simulink model "three_tank_open_loop"  (R2025b)
settings: Solver=ode4  StartTime=0.0  StopTime=20000  FixedStep=0.5  RelTol=1e-3
settings Model: Creator=user  LastModifiedBy=USER PC

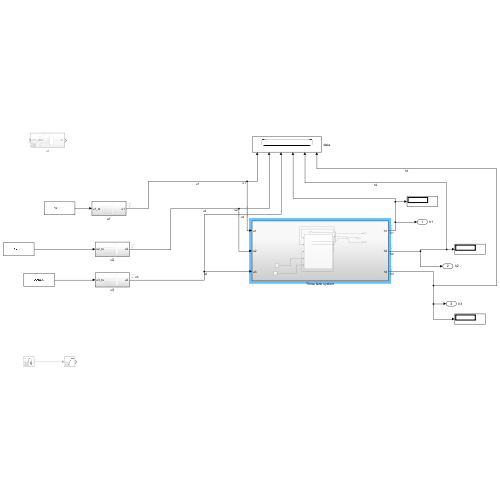
[thumbnail: Simulink's stored preview of the top-level diagram]
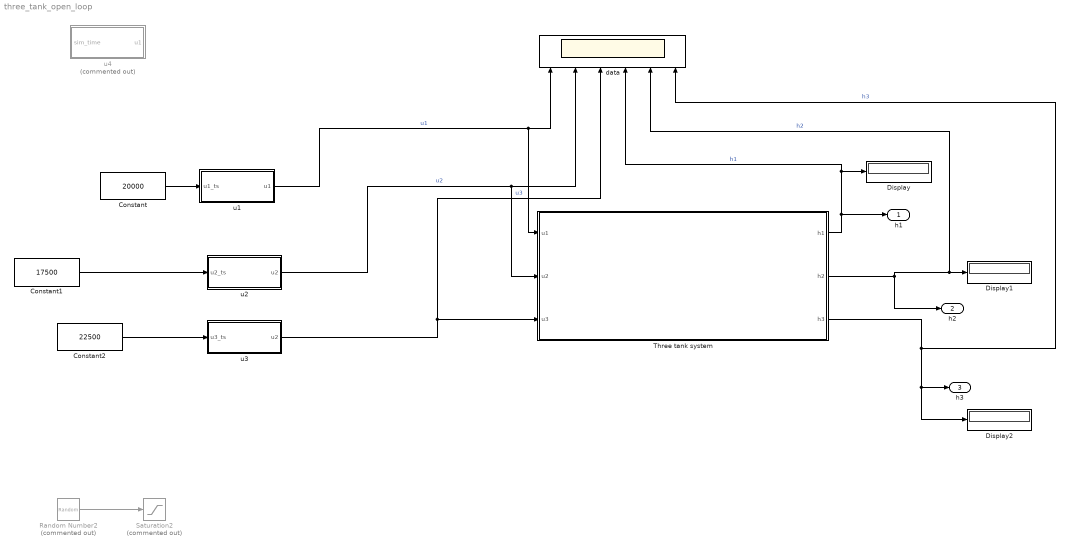
== system three_tank_open_loop ==
  Constant : Constant  Value=20000
  Constant1 : Constant  Value=17500
  Constant2 : Constant  Value=22500
  Display : Display
  Display1 : Display
  Display2 : Display
  Random Number2 : RandomNumber  Commented=on  Mean=0.2  Variance=0.01  Seed=1600  SampleTime=50
  Saturation2 : Saturate  Commented=on  UpperLimit=0.4  LowerLimit=0.01
  Three tank system : Subsystem
  data : Scope  NumInputPorts=6
      settings: ActiveDisplayString=5  Title=Tank 2 Height  ShowGrid=off  ActiveDisplayYMinimum=-4.7717687691549289  ActiveDisplayYMaximum=43.084803886371247  YLabel=Height (cm)  DataLoggingVariableName=dataset
  u1 : Subsystem
  u2 : Subsystem
  u3 : Subsystem
  u4 : Subsystem  Commented=on
  h1 : Outport
  h2 : Outport  Port=2
  h3 : Outport  Port=3
  wires:
  u3/1(u2) -> data/3, Three tank system/3(u3)  "u3"
  u2/1(u2) -> data/2, Three tank system/2(u2)  "u2"
  u1/1(u1) -> Three tank system/1(u1), data/1  "u1"
  Three tank system/3(h3) -> Display2/1, h3/1, data/6  "h3"
  Three tank system/2(h2) -> Display1/1, data/5, h2/1  "h2"
  Random Number2/1 -> Saturation2/1
  Three tank system/1(h1) -> h1/1, data/4, Display/1  "h1"
  Constant/1 -> u1/1(u1_ts)
  Constant1/1 -> u2/1(u2_ts)
  Constant2/1 -> u3/1(u3_ts)

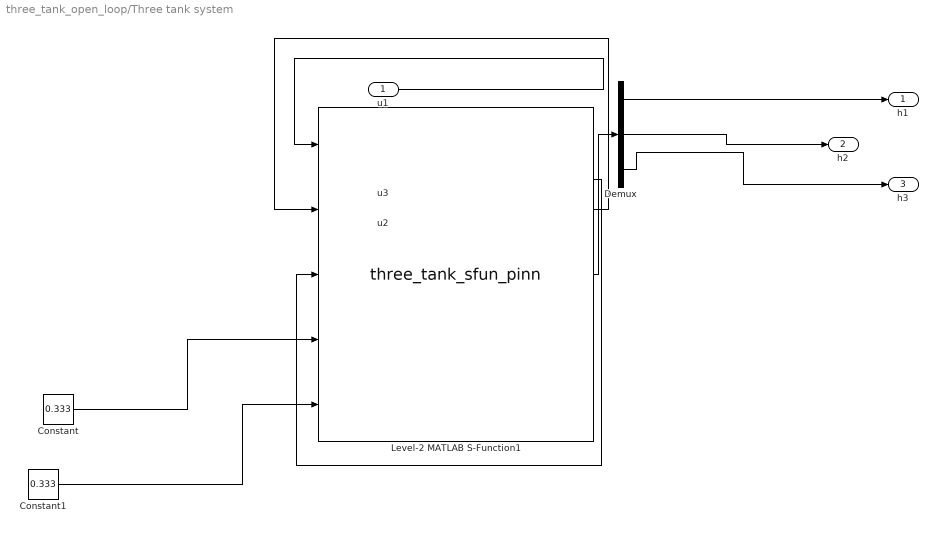
== system three_tank_open_loop/Three tank system ==
  u1 : Inport
  u2 : Inport  Port=2
  u3 : Inport  Port=3
  Constant : Constant  Value=0.333
  Constant1 : Constant  Value=0.333
  Demux : Demux  Outputs=3
  Level-2 MATLAB S-Function1 : M-S-Function  FunctionName=three_tank_sfun_pinn  Parameters=[5;5;5]
  h1 : Outport
  h2 : Outport  Port=2
  h3 : Outport  Port=3
  wires:
  u1/1 -> Level-2 MATLAB S-Function1/1
  u3/1 -> Level-2 MATLAB S-Function1/3
  u2/1 -> Level-2 MATLAB S-Function1/2
  Level-2 MATLAB S-Function1/1 -> Demux/1
  Demux/1 -> h1/1
  Demux/3 -> h3/1
  Demux/2 -> h2/1
  Constant/1 -> Level-2 MATLAB S-Function1/4
  Constant1/1 -> Level-2 MATLAB S-Function1/5

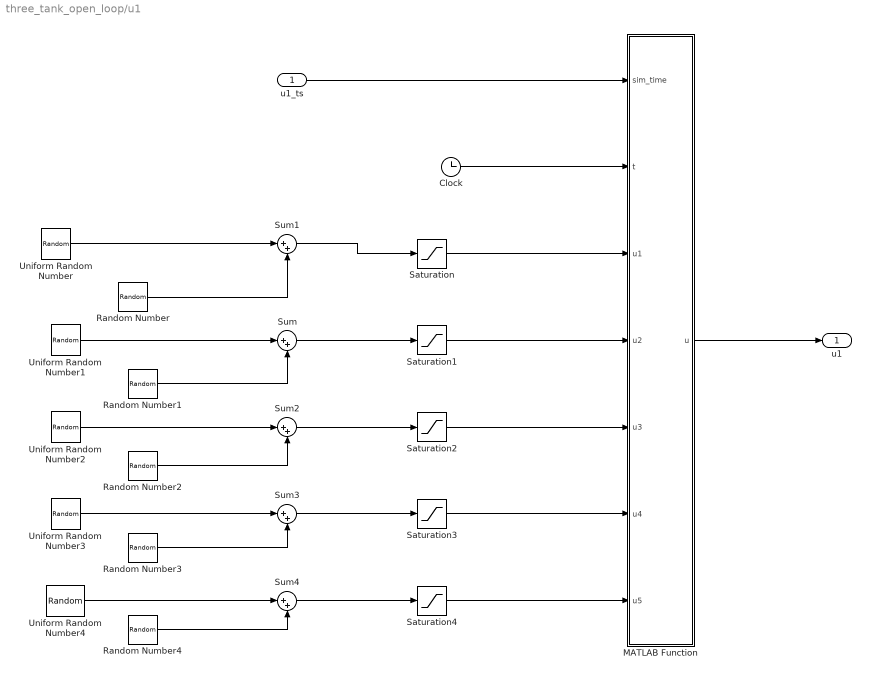
== system three_tank_open_loop/u1 ==
  u1_ts : Inport
  Clock : Clock
  MATLAB Function : MATLAB Function  TreatAsAtomicUnit=on
  Random Number : RandomNumber  Variance=0.05^2  Seed=122  SampleTime=1
  Random Number1 : RandomNumber  Variance=0.05^2  Seed=124  SampleTime=1
  Random Number2 : RandomNumber  Variance=0.05^2  Seed=126  SampleTime=1
  Random Number3 : RandomNumber  Variance=0.05^2  Seed=128  SampleTime=1
  Random Number4 : RandomNumber  Variance=0.05^2  Seed=130  SampleTime=1
  Saturation{,1..4} (5 alike) : Saturate  UpperLimit=148  LowerLimit=55
  Sum{,1..4} (5 alike) : Sum  Inputs=|++
  Uniform Random Number : UniformRandomNumber  Minimum=55  Maximum=148  Seed=121  SampleTime=20
  Uniform Random Number1 : UniformRandomNumber  Minimum=55  Maximum=148  Seed=123  SampleTime=40
  Uniform Random Number2 : UniformRandomNumber  Minimum=55  Maximum=148  Seed=125  SampleTime=60
  Uniform Random Number3 : UniformRandomNumber  Minimum=55  Maximum=148  Seed=127  SampleTime=80
  Uniform Random Number4 : UniformRandomNumber  Minimum=55  Maximum=148  Seed=129  SampleTime=100
  u1 : Outport
  wires:
  Clock/1 -> MATLAB Function/2(t)
  Saturation/1 -> MATLAB Function/3(u1)
  Saturation1/1 -> MATLAB Function/4(u2)
  Saturation2/1 -> MATLAB Function/5(u3)
  Saturation3/1 -> MATLAB Function/6(u4)
  Saturation4/1 -> MATLAB Function/7(u5)
  Random Number/1 -> Sum1/2
  Random Number1/1 -> Sum/2
  Random Number2/1 -> Sum2/2
  Random Number3/1 -> Sum3/2
  Random Number4/1 -> Sum4/2
  MATLAB Function/1(u) -> u1/1
  u1_ts/1 -> MATLAB Function/1(sim_time)
  Uniform Random Number4/1 -> Sum4/1
  Sum4/1 -> Saturation4/1
  Uniform Random Number3/1 -> Sum3/1
  Uniform Random Number2/1 -> Sum2/1
  Uniform Random Number1/1 -> Sum/1
  Uniform Random Number/1 -> Sum1/1
  Sum1/1 -> Saturation/1
  Sum/1 -> Saturation1/1
  Sum2/1 -> Saturation2/1
  Sum3/1 -> Saturation3/1

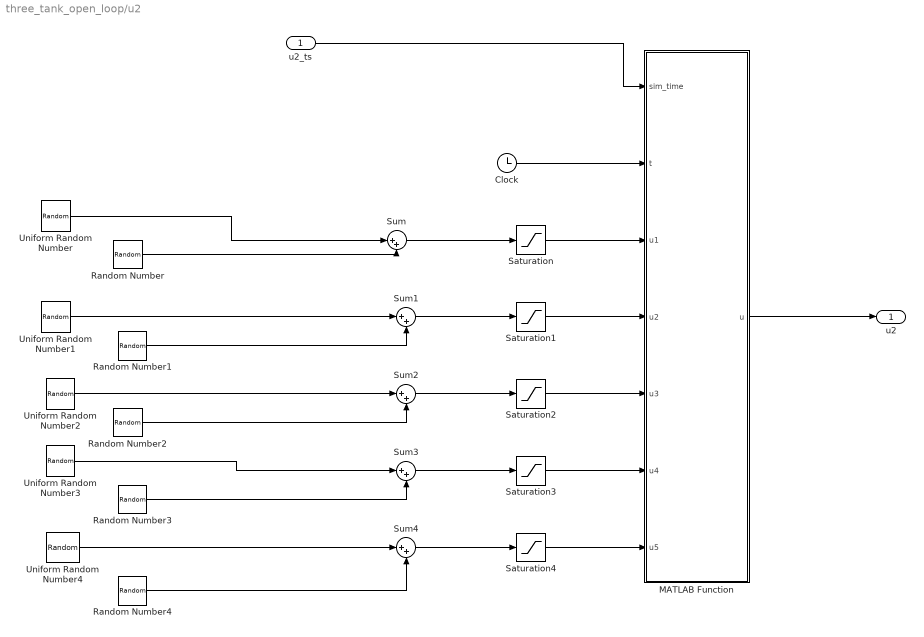
== system three_tank_open_loop/u2 ==
  u2_ts : Inport
  Clock : Clock
  MATLAB Function : MATLAB Function  TreatAsAtomicUnit=on
  Random Number : RandomNumber  Variance=0.01^2  Seed=233  SampleTime=1
  Random Number1 : RandomNumber  Variance=0.01^2  Seed=235  SampleTime=1
  Random Number2 : RandomNumber  Variance=0.01^2  Seed=238  SampleTime=1
  Random Number3 : RandomNumber  Variance=0.01^2  Seed=240  SampleTime=1
  Random Number4 : RandomNumber  Variance=0.01^2  Seed=242  SampleTime=1
  Saturation : Saturate  UpperLimit=1  LowerLimit=0.0
  Saturation1 : Saturate  UpperLimit=1.00  LowerLimit=0.0
  Saturation2 : Saturate  UpperLimit=1  LowerLimit=0.0
  Saturation3 : Saturate  UpperLimit=1  LowerLimit=0
  Saturation4 : Saturate  UpperLimit=1  LowerLimit=0
  Sum{,1..4} (5 alike) : Sum  Inputs=|++
  Uniform Random Number : UniformRandomNumber  Minimum=0.3  Maximum=0.6  Seed=233  SampleTime=20
  Uniform Random Number1 : UniformRandomNumber  Minimum=0.5  Seed=235  SampleTime=40
  Uniform Random Number2 : UniformRandomNumber  Minimum=0.2  Maximum=0.35  Seed=237  SampleTime=60
  Uniform Random Number3 : UniformRandomNumber  Minimum=0.4  Maximum=0.75  Seed=239  SampleTime=80
  Uniform Random Number4 : UniformRandomNumber  Minimum=0.25  Maximum=0.45  Seed=241  SampleTime=100
  u2 : Outport
  wires:
  Clock/1 -> MATLAB Function/2(t)
  Saturation/1 -> MATLAB Function/3(u1)
  Saturation1/1 -> MATLAB Function/4(u2)
  Saturation2/1 -> MATLAB Function/5(u3)
  Saturation3/1 -> MATLAB Function/6(u4)
  Saturation4/1 -> MATLAB Function/7(u5)
  Random Number/1 -> Sum/2
  Random Number1/1 -> Sum1/2
  Random Number2/1 -> Sum2/2
  Random Number3/1 -> Sum3/2
  Random Number4/1 -> Sum4/2
  MATLAB Function/1(u) -> u2/1
  u2_ts/1 -> MATLAB Function/1(sim_time)
  Uniform Random Number4/1 -> Sum4/1
  Sum4/1 -> Saturation4/1
  Uniform Random Number3/1 -> Sum3/1
  Sum3/1 -> Saturation3/1
  Sum2/1 -> Saturation2/1
  Uniform Random Number2/1 -> Sum2/1
  Uniform Random Number1/1 -> Sum1/1
  Uniform Random Number/1 -> Sum/1
  Sum1/1 -> Saturation1/1
  Sum/1 -> Saturation/1

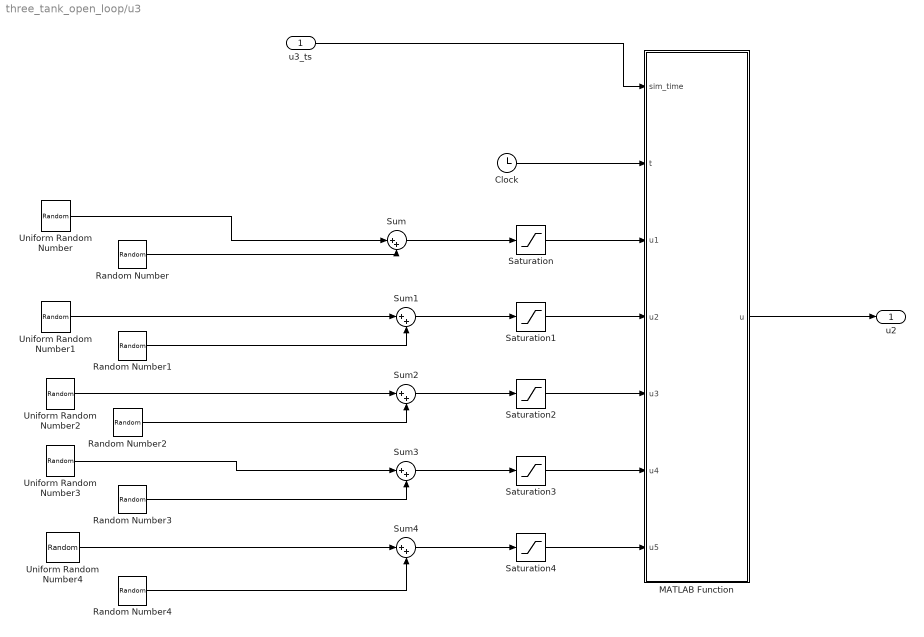
== system three_tank_open_loop/u3 ==
  u3_ts : Inport
  Clock : Clock
  MATLAB Function : MATLAB Function  TreatAsAtomicUnit=on
  Random Number : RandomNumber  Variance=0.01^2  Seed=312  SampleTime=1
  Random Number1 : RandomNumber  Variance=0.01^2  Seed=314  SampleTime=1
  Random Number2 : RandomNumber  Variance=0.01^2  Seed=316  SampleTime=1
  Random Number3 : RandomNumber  Variance=0.01^2  Seed=318  SampleTime=1
  Random Number4 : RandomNumber  Variance=0.01^2  Seed=320  SampleTime=1
  Saturation : Saturate  UpperLimit=1  LowerLimit=0
  Saturation{1..4} (4 alike) : Saturate  UpperLimit=1.0  LowerLimit=0.0
  Sum{,1..4} (5 alike) : Sum  Inputs=|++
  Uniform Random Number : UniformRandomNumber  Minimum=0.22  Maximum=0.45  Seed=311  SampleTime=20
  Uniform Random Number1 : UniformRandomNumber  Minimum=0.40  Maximum=0.85  Seed=312  SampleTime=40
  Uniform Random Number2 : UniformRandomNumber  Minimum=0.13  Maximum=0.26  Seed=315  SampleTime=60
  Uniform Random Number3 : UniformRandomNumber  Minimum=0.30  Maximum=0.58  Seed=317  SampleTime=80
  Uniform Random Number4 : UniformRandomNumber  Minimum=0.17  Maximum=0.34  Seed=319  SampleTime=100
  u2 : Outport
  wires:
  Clock/1 -> MATLAB Function/2(t)
  Saturation/1 -> MATLAB Function/3(u1)
  Saturation1/1 -> MATLAB Function/4(u2)
  Saturation2/1 -> MATLAB Function/5(u3)
  Saturation3/1 -> MATLAB Function/6(u4)
  Saturation4/1 -> MATLAB Function/7(u5)
  Random Number/1 -> Sum/2
  Random Number1/1 -> Sum1/2
  Random Number2/1 -> Sum2/2
  Random Number3/1 -> Sum3/2
  Random Number4/1 -> Sum4/2
  MATLAB Function/1(u) -> u2/1
  u3_ts/1 -> MATLAB Function/1(sim_time)
  Uniform Random Number4/1 -> Sum4/1
  Sum4/1 -> Saturation4/1
  Uniform Random Number3/1 -> Sum3/1
  Sum3/1 -> Saturation3/1
  Sum2/1 -> Saturation2/1
  Uniform Random Number2/1 -> Sum2/1
  Uniform Random Number1/1 -> Sum1/1
  Uniform Random Number/1 -> Sum/1
  Sum1/1 -> Saturation1/1
  Sum/1 -> Saturation/1

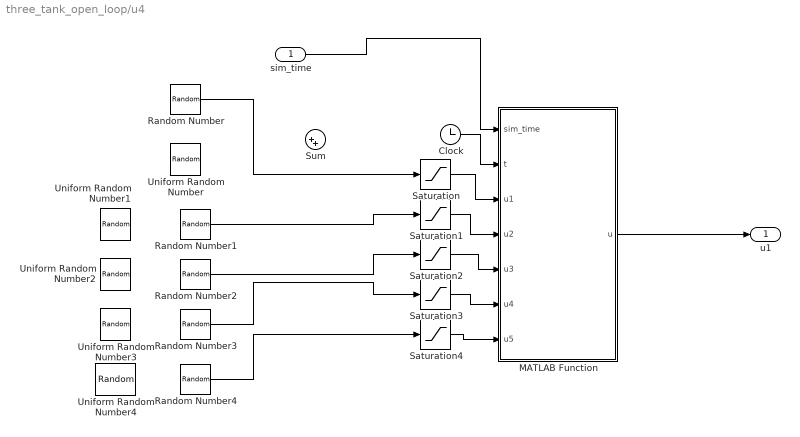
== system three_tank_open_loop/u4 ==
  sim_time : Inport
  Clock : Clock
  MATLAB Function : MATLAB Function  TreatAsAtomicUnit=on
  Random Number : RandomNumber  Mean=130  Variance=700  Seed=65374  SampleTime=20
  Random Number1 : RandomNumber  Mean=130  Variance=700  Seed=83984  SampleTime=15
  Random Number2 : RandomNumber  Mean=130  Variance=700  Seed=321194  SampleTime=10
  Random Number3 : RandomNumber  Mean=130  Variance=700  Seed=737284  SampleTime=5
  Random Number4 : RandomNumber  Mean=130  Variance=700  Seed=93884  SampleTime=3
  Saturation{,1..4} (5 alike) : Saturate  UpperLimit=167  LowerLimit=60
  Sum : Sum  Inputs=|++
  Uniform Random Number : UniformRandomNumber  Minimum=10  Maximum=200  Seed=213  SampleTime=20
  Uniform Random Number1 : UniformRandomNumber  Minimum=10  Maximum=200  Seed=2234  SampleTime=15
  Uniform Random Number2 : UniformRandomNumber  Minimum=10  Maximum=200  Seed=23422  SampleTime=10
  Uniform Random Number3 : UniformRandomNumber  Minimum=0  Maximum=200  Seed=42421  SampleTime=5
  Uniform Random Number4 : UniformRandomNumber  Minimum=10  Maximum=200  Seed=876  SampleTime=3
  u1 : Outport
  wires:
  Clock/1 -> MATLAB Function/2(t)
  Saturation/1 -> MATLAB Function/3(u1)
  Saturation1/1 -> MATLAB Function/4(u2)
  Saturation2/1 -> MATLAB Function/5(u3)
  Saturation3/1 -> MATLAB Function/6(u4)
  Saturation4/1 -> MATLAB Function/7(u5)
  Random Number/1 -> Saturation/1
  Random Number1/1 -> Saturation1/1
  Random Number2/1 -> Saturation2/1
  Random Number3/1 -> Saturation3/1
  Random Number4/1 -> Saturation4/1
  MATLAB Function/1(u) -> u1/1
  sim_time/1 -> MATLAB Function/1(sim_time)

== matlab function three_tank_open_loop/u1/MATLAB Function ==
  data: sim_time input; t input; u output; u1 input; u2 input; u3 input; u4 input; u5 input
function u = choose_signal(sim_time,t,u1,u2,u3,u4,u5)
u_opts = [u1,u2,u3,u4,u5];

stops = 0:round(sim_time/numel(u_opts)):sim_time;
u = u_opts(1);
for i = 1:numel(stops)-1
    if (t >= stops(i)) && (t <= stops(i+1))
        u = u_opts(i);
        break;
    end
end

== matlab function three_tank_open_loop/u2/MATLAB Function ==
  data: sim_time input; t input; u output; u1 input; u2 input; u3 input; u4 input; u5 input
function u = choose_signal(sim_time,t,u1,u2,u3,u4,u5)
u_opts = [u1,u2,u3,u4,u5];

stops = 0:round(sim_time/numel(u_opts)):sim_time;
u = u_opts(1);
for i = 1:numel(stops)-1
    if (t >= stops(i)) && (t <= stops(i+1))
        u = u_opts(i);
        break;
    end
end

== matlab function three_tank_open_loop/u4/MATLAB Function ==
  data: sim_time input; t input; u output; u1 input; u2 input; u3 input; u4 input; u5 input
function u = choose_signal(sim_time,t,u1,u2,u3,u4,u5)
u_opts = [u1,u2,u3,u4,u5];

stops = 0:round(sim_time/numel(u_opts)):sim_time;
u = u_opts(1);
for i = 1:numel(stops)-1
    if (t >= stops(i)) && (t <= stops(i+1))
        u = u_opts(i);
        break;
    end
end

== matlab function three_tank_open_loop/u3/MATLAB Function ==
  data: sim_time input; t input; u output; u1 input; u2 input; u3 input; u4 input; u5 input
function u = choose_signal(sim_time,t,u1,u2,u3,u4,u5)
u_opts = [u1,u2,u3,u4,u5];

stops = 0:round(sim_time/numel(u_opts)):sim_time;
u = u_opts(1);
for i = 1:numel(stops)-1
    if (t >= stops(i)) && (t <= stops(i+1))
        u = u_opts(i);
        break;
    end
end
